simulink model "sim_lw8"  (R2025a)
settings: Solver=VariableStepAuto  StartTime=0.0  StopTime=10  RelTol=1e-3
values from neighbouring files (symbols this model uses):
  b = 0.2    [lw8_1.m]
  c = 0.15    [lw8_1.m]
  C_vx1 = 59    [lw8_2.m]
  C_vx2 = 5.9    [lw8_2.m]
  C_vy1 = 62    [lw8_2.m]
  C_vy2 = 6.2    [lw8_2.m]
  C_wy1 = 96    [lw8_1.m]
  C_wy2 = 9.6    [lw8_1.m]
  C_wz1 = 98    [lw8_1.m]
  C_wz2 = 9.8    [lw8_1.m]
  g = 9.81    [lw8_1.m]
  Jy = 128    [lw8_1.m]
  K_dv = 15    [lw8_1.m]    (also in lw8_2.m)
  lambda11 = 98    [lw8_2.m]
  lambda22 = 104    [lw8_2.m]
  lambda55 = 126    [lw8_1.m]
  lambda66 = 125    [lw8_1.m]
  m = 110    [lw8_1.m]    (also in lw8_2.m)
  ro = 1025    [lw8_1.m]
  T_dv = 0.15    [lw8_1.m]    (also in lw8_2.m)
  V = 0.2    [lw8_1.m]
settings Model: Creator=user  LastModifiedBy=user

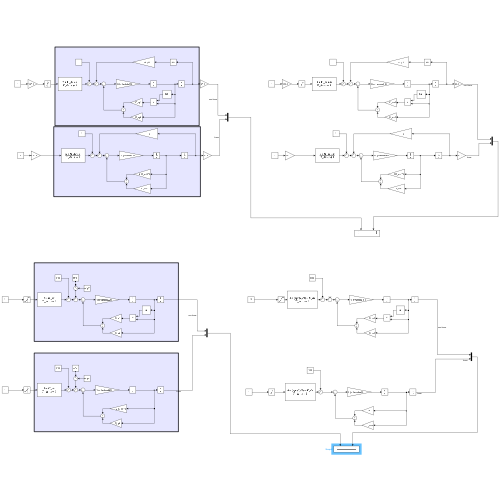
[thumbnail: Simulink's stored preview of the top-level diagram]
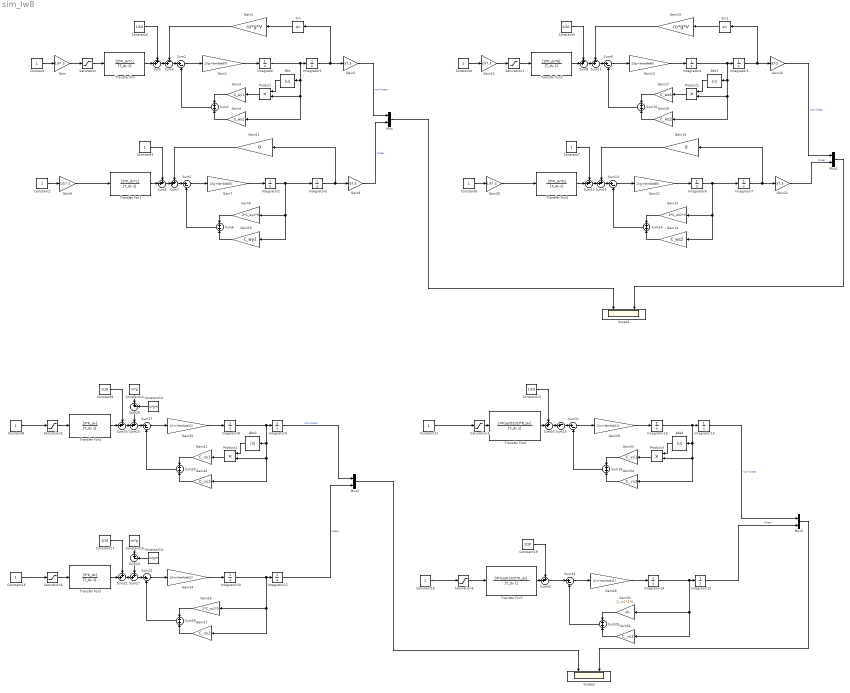
== system sim_lw8 ==
  Abs{,1..3} (4 alike) : Abs  SaturateOnIntegerOverflow=off
  Constant{,2..4,6..8,12,16,18} (10 alike) : Constant
  Constant{1,5,9,13,17,19} (6 alike) : Constant  Value=1/10
  Constant10 : Constant  Value=ro*g*V
  Constant11 : Constant  Value=m*g
  Constant14 : Constant  Value=ro*g*V
  Constant15 : Constant  Value=m*g
  Gain{,6,12,20} (4 alike) : Gain  Gain=1/57.3
  Gain1 : Gain  Gain=1/(Jy+lambda55)
  Gain10 : Gain  Gain=C_wy2
  Gain11 : Gain  Gain=0
  Gain13 : Gain  Gain=1/(Jy+lambda66)
  Gain14 : Gain  Gain=C_wz2
  Gain15 : Gain  Gain=0
  Gain{2,8,16,22} (4 alike) : Gain  Gain=57.3
  Gain17 : Gain  Gain=C_wz1
  Gain18 : Gain  Gain=C_wz2
  Gain19 : Gain  Gain=ro*g*V
  Gain21 : Gain  Gain=1/(Jy+lambda66)
  Gain23 : Gain  Gain=2*C_wz1*0
  Gain24 : Gain  Gain=1/(m+lambda22)
  Gain25 : Gain  Gain=1/(m+lambda22)
  Gain26 : Gain  Gain=2*C_vy1*0
  Gain27 : Gain  Gain=C_vy2
  Gain28 : Gain  Gain=1/(m+lambda11)
  Gain29 : Gain  Gain=1/(m+lambda11)
  Gain3 : Gain  Gain=C_wy1
  Gain30 : Gain  Gain=C_vx1*2*0
  Gain31 : Gain  Gain=C_vx2
  Gain33 : Gain  Gain=C_vx1
  Gain34 : Gain  Gain=C_vx2
  Gain4 : Gain  Gain=C_wy2
  Gain41 : Gain  Gain=C_vy1
  Gain42 : Gain  Gain=C_vy2
  Gain5 : Gain  Gain=ro*g*V
  Gain7 : Gain  Gain=1/(Jy+lambda55)
  Gain9 : Gain  Gain=2*C_wy1*0
  Integrator{,1..15} (16 alike) : Integrator
  Mux{,1..3} (4 alike) : Mux  Inputs=2
  Product{,1..3} (4 alike) : Product
  Saturation{,1..5} (6 alike) : Saturate  UpperLimit=10  LowerLimit=10
  Scope1 : Scope  NumInputPorts=2
      settings: ActiveDisplayYMinimum=-1.4384433356618187  ActiveDisplayYMaximum=12.945990020956371
  Scope2 : Scope  NumInputPorts=2
      settings: ActiveDisplayYMinimum=-118.30071463310595  ActiveDisplayYMaximum=13.14452384812288
  Sin : Trigonometry
  Sin1 : Trigonometry
  Sum{,4,7..8,12,15..16,21,25,27,30,32} (12 alike) : Sum  Inputs=++|
  Sum{1,5,9,13,17,20,22..23,31,33} (10 alike) : Sum  Inputs=|+-
  Sum{2,6,10,14,18,24,26,28} (8 alike) : Sum
  Sum11 : Sum  Inputs=-+|
  Sum19 : Sum  Inputs=-+|
  Sum3 : Sum  Inputs=-+|
  Transfer Fcn : TransferFcn  Numerator=[2*K_dv*c]  Denominator=[T_dv 1]
  Transfer Fcn1 : TransferFcn  Numerator=[2*K_dv*c]  Denominator=[T_dv 1]
  Transfer Fcn2 : TransferFcn  Numerator=[3*K_dv*b]  Denominator=[T_dv 1]
  Transfer Fcn3 : TransferFcn  Numerator=[3*K_dv*b]  Denominator=[T_dv 1]
  Transfer Fcn4 : TransferFcn  Numerator=[3*K_dv]  Denominator=[T_dv 1]
  Transfer Fcn5 : TransferFcn  Numerator=[3*K_dv]  Denominator=[T_dv 1]
  Transfer Fcn6 : TransferFcn  Numerator=[4*(sqrt(2)/2)*K_dv]  Denominator=[T_dv 1]
  Transfer Fcn7 : TransferFcn  Numerator=[4*(sqrt(2)/2)*K_dv]  Denominator=[T_dv 1]
  wires:
  Constant/1 -> Gain/1
  Gain/1 -> Saturation/1
  Saturation/1 -> Transfer Fcn/1
  Transfer Fcn/1 -> Sum/2
  Constant1/1 -> Sum/1
  Sum1/1 -> Gain1/1
  Gain1/1 -> Integrator/1
  Integrator/1 -> Gain4/1, Product/2, Abs/1, Integrator1/1
  Integrator1/1 -> Sin/1, Gain2/1
  Gain2/1 -> Mux/1  "non-linear"
  Abs/1 -> Product/1
  Product/1 -> Gain3/1
  Gain3/1 -> Sum2/1
  Gain4/1 -> Sum2/2
  Sum2/1 -> Sum1/2
  Sum/1 -> Sum3/2
  Sum3/1 -> Sum1/1
  Gain5/1 -> Sum3/1
  Sin/1 -> Gain5/1
  Sum4/1 -> Sum7/2
  Sum7/1 -> Sum5/1
  Integrator3/1 -> Gain11/1, Gain8/1
  Sum6/1 -> Sum5/2
  Gain9/1 -> Sum6/1
  Integrator2/1 -> Integrator3/1, Gain10/1, Gain9/1
  Gain10/1 -> Sum6/2
  Gain11/1 -> Sum7/1
  Gain7/1 -> Integrator2/1
  Sum5/1 -> Gain7/1
  Transfer Fcn1/1 -> Sum4/2
  Gain6/1 -> Transfer Fcn1/1
  Constant2/1 -> Gain6/1
  Constant3/1 -> Sum4/1
  Gain8/1 -> Mux/2  "linear"
  Gain20/1 -> Transfer Fcn3/1
  Sum11/1 -> Sum9/1
  Sin1/1 -> Gain19/1
  Product1/1 -> Gain17/1
  Gain18/1 -> Sum10/2
  Gain19/1 -> Sum11/1
  Gain13/1 -> Integrator4/1
  Sum9/1 -> Gain13/1
  Integrator6/1 -> Integrator7/1, Gain14/1, Gain23/1
  Constant6/1 -> Gain20/1
  Integrator7/1 -> Gain15/1, Gain22/1
  Sum14/1 -> Sum13/2
  Transfer Fcn3/1 -> Sum12/2
  Gain17/1 -> Sum10/1
  Gain23/1 -> Sum14/1
  Gain15/1 -> Sum15/1
  Abs1/1 -> Product1/1
  Gain14/1 -> Sum14/2
  Sum10/1 -> Sum9/2
  Sum8/1 -> Sum11/2
  Sum15/1 -> Sum13/1
  Integrator5/1 -> Sin1/1, Gain16/1
  Transfer Fcn2/1 -> Sum8/2
  Sum12/1 -> Sum15/2
  Gain12/1 -> Saturation1/1
  Constant7/1 -> Sum12/1
  Saturation1/1 -> Transfer Fcn2/1
  Constant4/1 -> Gain12/1
  Gain21/1 -> Integrator6/1
  Integrator4/1 -> Gain18/1, Product1/2, Abs1/1, Integrator5/1
  Constant5/1 -> Sum8/1
  Sum13/1 -> Gain21/1
  Gain16/1 -> Mux1/1  "non-linear"
  Gain22/1 -> Mux1/2  "linear"
  Mux1/1 -> Scope1/2
  Mux/1 -> Scope1/1
  Constant13/1 -> Sum30/1
  Abs3/1 -> Product3/1
  Sum18/1 -> Sum31/2
  Transfer Fcn6/1 -> Sum30/2
  Sum30/1 -> Sum19/2
  Saturation3/1 -> Transfer Fcn6/1
  Constant12/1 -> Saturation3/1
  Gain33/1 -> Sum18/1
  Product3/1 -> Gain33/1
  Gain29/1 -> Integrator12/1
  Gain34/1 -> Sum18/2
  Sum25/1 -> Sum17/1
  Mux3/1 -> Scope2/2
  Gain42/1 -> Sum24/2
  Integrator15/1 -> Mux3/2  "linear"
  Product2/1 -> Gain41/1
  Integrator9/1 -> Mux2/1  "non-linear"
  Integrator13/1 -> Mux3/1  "non-linear"
  Sum31/1 -> Gain29/1
  Sum20/1 -> Sum25/1
  Gain25/1 -> Integrator8/1
  Sum17/1 -> Gain25/1
  Gain41/1 -> Sum24/1
  Abs2/1 -> Product2/1
  Integrator12/1 -> Gain34/1, Product3/2, Abs3/1, Integrator13/1
  Sum24/1 -> Sum17/2
  Sum16/1 -> Sum25/2
  Transfer Fcn4/1 -> Sum16/2
  Constant8/1 -> Saturation2/1
  Saturation2/1 -> Transfer Fcn4/1
  Integrator8/1 -> Gain42/1, Product2/2, Abs2/1, Integrator9/1
  Sum19/1 -> Sum31/1
  Constant9/1 -> Sum16/1
  Mux2/1 -> Scope2/1
  Constant10/1 -> Sum20/2
  Constant11/1 -> Sum20/1
  Gain24/1 -> Integrator10/1
  Sum22/1 -> Gain24/1
  Gain27/1 -> Sum26/2
  Integrator10/1 -> Gain27/1, Gain26/1, Integrator11/1
  Constant15/1 -> Sum23/1
  Constant17/1 -> Sum21/1
  Saturation4/1 -> Transfer Fcn5/1
  Transfer Fcn5/1 -> Sum21/2
  Sum27/1 -> Sum22/1
  Integrator11/1 -> Mux2/2  "linear"
  Gain26/1 -> Sum26/1
  Sum23/1 -> Sum27/1
  Sum26/1 -> Sum22/2
  Constant14/1 -> Sum23/2
  Sum21/1 -> Sum27/2
  Constant16/1 -> Saturation4/1
  Gain28/1 -> Integrator14/1
  Sum32/1 -> Sum33/1
  Integrator14/1 -> Gain30/1, Gain31/1, Integrator15/1
  Transfer Fcn7/1 -> Sum32/2
  Constant19/1 -> Sum32/1
  Constant18/1 -> Saturation5/1
  Saturation5/1 -> Transfer Fcn7/1
  Sum28/1 -> Sum33/2
  Sum33/1 -> Gain28/1
  Gain30/1 -> Sum28/1
  Gain31/1 -> Sum28/2
